simulink model "sfWindTurbine"  (R2025b)
settings: Solver=ode23t  StartTime=0.0  StopTime=simT  RelTol=1e-3  AbsTol=1e-3
PreLoadFcn:
  | load sfWindTurbineParameters.mat
values from neighbouring files (symbols this model uses):
  actuatorRampRate = 20    [sfWindTurbineParameters.mat]
  airDensity = 1.15    [sfWindTurbineParameters.mat]
  carrierShaftInertia = 10    [sfWindTurbineParameters.mat]
  controllerTimeConstant = 2    [sfWindTurbineParameters.mat]
  cp = [1e-05 1e-05 1e-05 1e-05 1e-05 1e-05 1e-05 1e-05 1e-05 1e-05 1e-05 1e-05 ... (3015 elements, 15x201)]    [sfWindTurbineParameters.mat]
  Derating = [12 13 14 15 16 17 18 19 20 1 4 7 ... (18 elements, 9x2)]    [sfWindTurbineParameters.mat]
  firstStepTeethRatio = 3.05    [sfWindTurbineParameters.mat]
  generatorEfficiency = 100    [sfWindTurbineParameters.mat]
  generatorInertia = 200    [sfWindTurbineParameters.mat]
  generatorLumpedInductance = 0.0001916    [sfWindTurbineParameters.mat]
  generatorLumpedResistance = 0.0027    [sfWindTurbineParameters.mat]
  gridFrequency = 60    [sfWindTurbineParameters.mat]
  iGenerationGain = 1    [sfWindTurbineParameters.mat]
  maxPitchAngle = 25    [sfWindTurbineParameters.mat]
  minPitchAngle = 1    [sfWindTurbineParameters.mat]
  mpptOmega = [502.335 613.965 753.5025 865.1325 1004.67 1116.3 1200.0225 1200.0225 1200.0225]    [sfWindTurbineParameters.mat]
  mpptPower = [0.0596400180021 0.116487570967 0.201285060757 0.319665137738 0.477120144017 0.679427108153 0.931130687114 1.22525336077 1.55330342875]    [sfWindTurbineParameters.mat]
  mpptWindSpeed = [4 5 6 7 8 9 10 11 12]    [sfWindTurbineParameters.mat]
  pGenerationGain = 100    [sfWindTurbineParameters.mat]
  pGeneratorBrakeLimit = 0.5    [sfWindTurbineParameters.mat]
  pitch = [1 3 5 7 9 11 13 15 17 19 21 23 ... (15 elements, 1x15)]    [sfWindTurbineParameters.mat]
  pitchBrakeAngle = 95    [sfWindTurbineParameters.mat]
  ringSunTeethRatio = 6    [sfWindTurbineParameters.mat]
  rotorBladeInertia = 3963845    [sfWindTurbineParameters.mat]
  secondStepTeethRatio = 3.05    [sfWindTurbineParameters.mat]
  simT = 800    [sfWindTurbineParameters.mat]
  stepShaftInertia = 10    [sfWindTurbineParameters.mat]
  TSR = [0 0.1 0.2 0.3 0.4 0.5 0.6 0.7 0.8 0.9 1 1.1 ... (201 elements, 1x201)]    [sfWindTurbineParameters.mat]
  turbineRadius = 35.25    [sfWindTurbineParameters.mat]
  turbineRatedPower = 1.5    [sfWindTurbineParameters.mat]
  vWindCutOut = 20    [sfWindTurbineParameters.mat]
  wAtGeneratorRatedPower = 1227.93    [sfWindTurbineParameters.mat]
  wGeneratorBrakeLimit = 0.5    [sfWindTurbineParameters.mat]
libraries: simulink x6, slpidlib x1, SignalEditorBlockLib x1
Description:
  | Wind Turbine
settings Model: PauseTimes=599  Creator=The MathWorks, Inc.  LastModifiedBy=The MathWorks, Inc.
settings SolverCC: AutoScaleAbsTol=off  MaxConsecutiveMinStep=5  AlgebraicLoopSolver=TrustRegion  MaxZcPerStep=1.0
settings DataIOCC: SaveOutput=off  DSMLogging=off  SaveTime=off  ReturnWorkspaceOutputs=off  SignalLoggingName=logsout_sscv_wind_turbine
settings OptimizationCC: ReuseModelBlockBuffer=off
settings DebuggingCC: UnconnectedInputMsg=warning  UnconnectedOutputMsg=warning  UnconnectedLineMsg=warning
settings ModelReferenceCC: EnableRefExpFcnMdlSchedulingChecks=on
settings RTWCC: GPUComputeCapability=3.5  DLArmComputeVersion=19.05
settings SimscapeCC: SimscapeLogType=all  SimscapeLogSimulationStatistics=on  SimscapeLogName=simlog_sscv_wind_turbine  SimscapeLogDataHistory=10000000.0
settings ConfigComp: PLC_FoldFBCallOutputVar=off  PLC_RemoveUnusedSSMethodCallArguments=off  PLC_ActiveTab=0.0  PLC_UseCallOutputArgSyntax=off  PLC_TargetIDE=codesys35  PLC_EnableUnsignedAndDoubleTypes=off  PLC_RollThreshold=5.0  PLC_EnableUDTSplitting=off  PLC_MultiTBSigbuilderTimeRange=off  PLC_MaxFieldsInUDT=500.0  PLC_EnableStringLiteralTB=on  PLC_InlineEnumCastFunction=off  PLC_Enable64bitIntSupport=off  PLC_RTWMaxIdLength=31.0

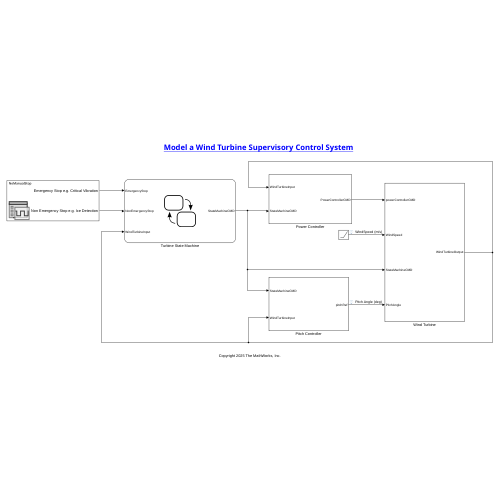
[thumbnail: Simulink's stored preview of the top-level diagram]
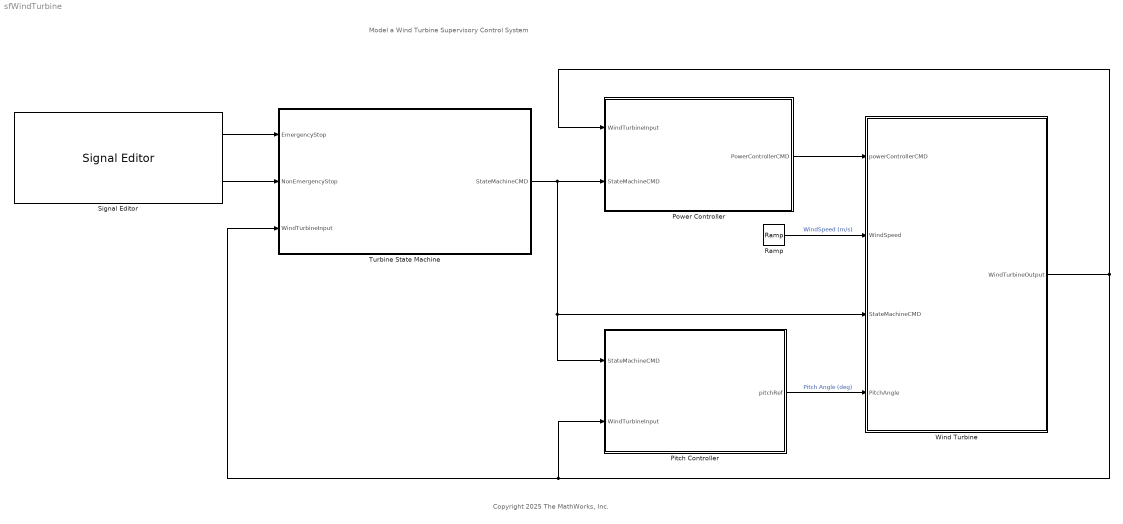
== system sfWindTurbine ==
  note: Model a Wind Turbine Supervisory Control System
  note: Copyright 2025 The MathWorks, Inc.
  Pitch Controller : Subsystem
  Power Controller : Subsystem
  Ramp : simulink/Sources/Ramp  slope=(vWindCutOut+2)/simT  start=0  InitialOutput=0
  Signal Editor : SignalEditorBlockLib/Signal Editor  FileName=ManualStopSignal.mat  ActiveScenario=NoManualStop  ActiveSignal=Emergency Stop e.g. Critical Vibration  IsBus=off  OutputBusObjectStr=Bus: BusObject  SampleTime=0  Interpolate=off  ZeroCross=off  OutputAfterFinalValue=Setting to zero  Unit=inherit  PreserveSignalName=on  ApplySigPropsToAllScenarios=on  ApplySigPropsToAllSignals=off  SignalPropertySource=Dialog parameters
  Turbine State Machine : Stateflow chart  TreatAsAtomicUnit=on
  Wind Turbine : Subsystem
  wires:
  Turbine State Machine/1(StateMachineCMD) -> Pitch Controller/1(StateMachineCMD), Wind Turbine/3(StateMachineCMD), Power Controller/2(StateMachineCMD)
  Pitch Controller/1(pitchRef) -> Wind Turbine/4(PitchAngle)  "Pitch Angle (deg)"
  Ramp/1 -> Wind Turbine/2(WindSpeed)  "WindSpeed (m/s)"
  Power Controller/1(PowerControllerCMD) -> Wind Turbine/1(powerControllerCMD)
  Wind Turbine/1(WindTurbineOutput) -> Power Controller/1(WindTurbineInput), Pitch Controller/2(WindTurbineInput), Turbine State Machine/3(WindTurbineInput)
  Signal Editor/1 -> Turbine State Machine/1(EmergencyStop)
  Signal Editor/2 -> Turbine State Machine/2(NonEmergencyStop)

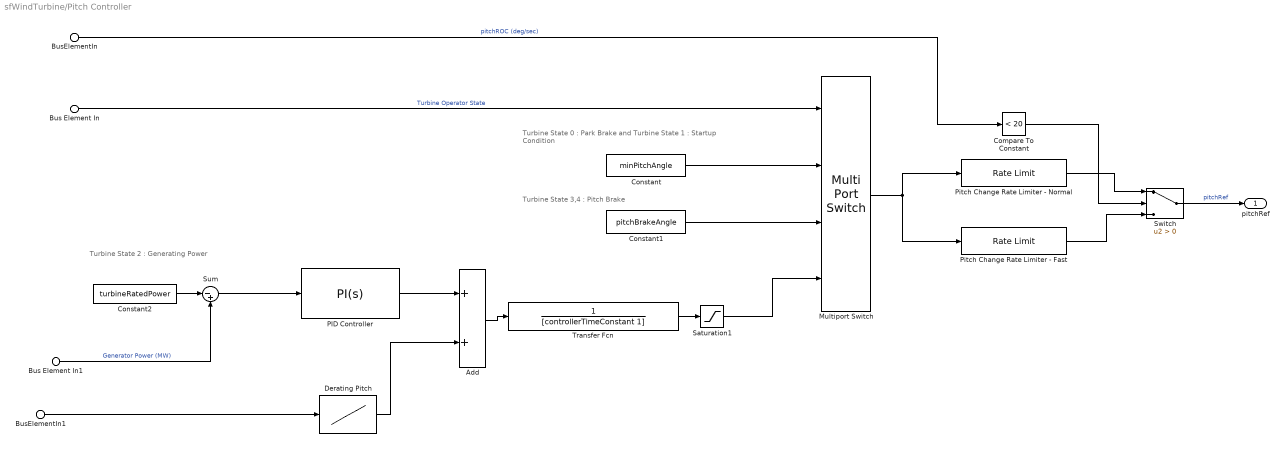
== system sfWindTurbine/Pitch Controller ==
  note: Turbine State 2 : Generating Power
  note: Turbine State 0 : Park Brake and
      | Turbine State 1 : Startup Condition
  note: Turbine State 3,4 : Pitch Brake
  Bus Element In : Inport  PortName=StateMachineCMD  Element=turbineState
  BusElementIn : Inport  PortName=StateMachineCMD  Element=pitchROC
  Bus Element In1 : Inport  Port=2  PortName=WindTurbineInput  Element=GeneratorPower
  BusElementIn1 : Inport  Port=2  PortName=WindTurbineInput  Element=WindSpeed
  Add : Sum  Inputs=2
  Compare To Constant : simulink/Logic and Bit Operations/Compare To Constant  relop=<  const=20  OutDataTypeStr=boolean
  Constant : Constant  Value=minPitchAngle
  Constant1 : Constant  Value=pitchBrakeAngle
  Constant2 : Constant  Value=turbineRatedPower
  Derating Pitch : Lookup_n-D  NumberOfTableDimensions=1  BreakpointsForDimension1=Derating(:,1)  Table=Derating(:,2)-minPitchAngle  InternalRulePriority=Speed  RndMeth=Simplest
  Multiport Switch : MultiPortSwitch  DataPortOrder=Specify indices  DataPortIndices={[0,1],[3,4],2}  SaturateOnIntegerOverflow=off  InputSameDT=off
  PID Controller : slpidlib/PID Controller  Controller=PI  Form=Parallel  TimeDomain=Continuous-time  UseExternalTs=off  SampleTime=-1  IntegratorMethod=Forward Euler  FilterMethod=Forward Euler  ControllerParametersSource=internal  P=pGenerationGain  I=iGenerationGain  UseKiTs=off  D=0  UseExternalDerivativeSource=off  N=100  UseFilter=on  TunerSelectOption=Transfer Function Based (PID Tuner App)  InitialConditionSource=internal  InitialConditionForIntegrator=1  InitialConditionForFilter=0  DifferentiatorICPrevScaledInput=0  ExternalReset=none  TrackingMode=off  Kt=1  LimitOutput=on  SatLimitsSource=internal  UpperSaturationLimit=maxPitchAngle  LowerSaturationLimit=minPitchAngle  LinearizeAsGain=on  AntiWindupMode=clamping  Kb=1  LimitIntegrator=off  UpperIntegratorSaturationLimit=inf  LowerIntegratorSaturationLimit=-inf  POutMin=[]  POutMax=[]  IOutMin=[]  IOutMax=[]  DOutMin=[]  DOutMax=[]  NOutMin=[]  NOutMax=[]  SumOutMin=[]  SumOutMax=[]  SaturationOutMin=[]  SaturationOutMax=[]  PParamMin=[]  PParamMax=[]  IParamMin=[]  IParamMax=[]  DParamMin=[]  DParamMax=[]  NParamMin=[]  NParamMax=[]  KbParamMin=[]  KbParamMax=[]  KtParamMin=[]  KtParamMax=[]  KbOutMin=[]  KbOutMax=[]  KtOutMin=[]  KtOutMax=[]  IntegratorOutMin=[]  IntegratorOutMax=[]  FilterOutMin=[]  FilterOutMax=[]  SumI1OutMin=[]  SumI1OutMax=[]  SumI2OutMin=[]  SumI2OutMax=[]  SumI3OutMin=[]  SumI3OutMax=[]  SumI4OutMin=[]  SumI4OutMax=[]  SumDOutMin=[]  SumDOutMax=[]  DifferentiatorOutMin=[]  DifferentiatorOutMax=[]  FilterDiffOutCoefMin=[]  FilterDiffOutCoefMax=[]  ReciprocalOutMin=[]  ReciprocalOutMax=[]  SumDenOutMin=[]  SumDenOutMax=[]  SumNumOutMin=[]  SumNumOutMax=[]  DivideOutMin=[]  DivideOutMax=[]  UdiffTsProdOutMin=[]  UdiffTsProdOutMax=[]  NTsProdOutMin=[]  NTsProdOutMax=[]  UintegralTsProdOutMin=[]  UintegralTsProdOutMax=[]  UngainTsProdOutMin=[]  UngainTsProdOutMax=[]  ClampingZeroOutDataTypeStr=Inherit: Inherit via back propagation  ClampingZeroOutMin=[]  ClampingZeroOutMax=[]  FilterDenConstantOutDataTypeStr=Inherit: Inherit via back propagation  FilterDenConstantOutMin=[]  FilterDenConstantOutMax=[]  PCopyOutDataTypeStr=Inherit: Inherit via back propagation  PCopyOutMin=[]  PCopyOutMax=[]  NCopyOutDataTypeStr=Inherit: Inherit via back propagation  NCopyOutMin=[]  NCopyOutMax=[]  IntegratorContinuousStateAttributes=''  IntegratorStateMustResolveToSignalObject=off  IntegratorRTWStateStorageClass=Auto  FilterContinuousStateAttributes=''  FilterStateMustResolveToSignalObject=off  FilterRTWStateStorageClass=Auto  ParallelPVariant=InternalParameters  IdealPVariant=Disabled  IVariant=InternalParameters  DVariant=Disabled  IntegratorVariant=Continuous  SatVariant=Enabled  AWVariant=ContClampingParallel  PCopyVariant=Disabled  TRVariant=Disabled  FdbkBlocksVariant=Forward  IdealPFdbkVariant=Disabled  SatFdbkVariant=Disabled  DerivativeFilterVariant=Disabled  NVariant=Disabled  NCopyVariant=Disabled_SignalSpec  FilterICVariant=Disabled  IntegratorICVariant=InternalICs  ExternalResetVariant=Disabled  TRSumVariant=Passthrough  SumFdbkVariant=Disabled  SumVariant=Sum_PI  TsampFilterVariant=InternalTs  TsampNgainVariant=Passthrough  TsampIntegralVariant=Disabled_SignalSpec  ExternalSaturationOutDataTypeStr=Inherit: Same as second input  DerivativeSourceVariant=Disabled  PreIntVariant=InternalPreInt
      settings: AttributesFormatString=|
      | %<AntiWindupMode>
      | %<I>
      | %<P>
      | %<UpperSaturationLimit>
      | %<LowerSaturationLimit>
  Pitch Change Rate Limiter - Fast : RateLimiter  RisingSlewLimit=actuatorRampRate  FallingSlewLimit=-actuatorRampRate  SampleTimeMode=inherited
  Pitch Change Rate Limiter - Normal : RateLimiter  RisingSlewLimit=actuatorRampRate/4  FallingSlewLimit=-actuatorRampRate/4  SampleTimeMode=inherited
  Saturation1 : Saturate  UpperLimit=maxPitchAngle  LowerLimit=minPitchAngle
  Sum : Sum  Inputs=|-+
  Switch : Switch  Criteria=u2 > Threshold  SaturateOnIntegerOverflow=off  InputSameDT=off
  Transfer Fcn : TransferFcn  Denominator=[controllerTimeConstant 1]
  pitchRef : Outport
  wires:
  Pitch Change Rate Limiter - Normal/1 -> Switch/1
  Derating Pitch/1 -> Add/2
  Compare To Constant/1 -> Switch/2
  Pitch Change Rate Limiter - Fast/1 -> Switch/3
  Multiport Switch/1 -> Pitch Change Rate Limiter - Fast/1, Pitch Change Rate Limiter - Normal/1
  Constant/1 -> Multiport Switch/2
  Saturation1/1 -> Multiport Switch/4
  PID Controller/1 -> Add/1
  Constant1/1 -> Multiport Switch/3
  Transfer Fcn/1 -> Saturation1/1
  Add/1 -> Transfer Fcn/1
  Constant2/1 -> Sum/1
  Sum/1 -> PID Controller/1
  Switch/1 -> pitchRef/1  "pitchRef"
  BusElementIn/1 -> Compare To Constant/1  "pitchROC (deg/sec)"
  Bus Element In1/1 -> Sum/2  "Generator Power (MW)"
  Bus Element In/1 -> Multiport Switch/1  "Turbine Operator State"
  BusElementIn1/1 -> Derating Pitch/1

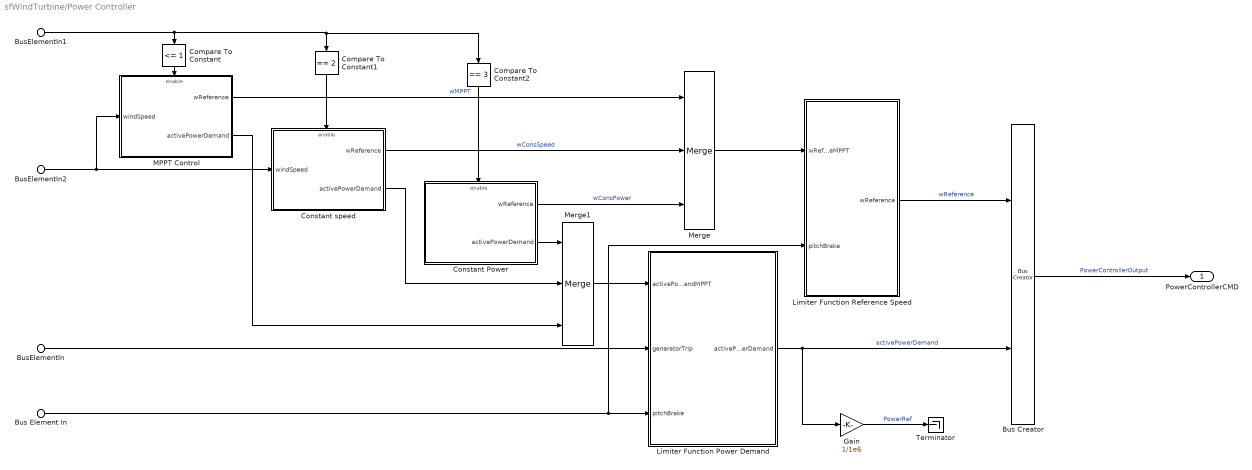
== system sfWindTurbine/Power Controller ==
  BusElementIn2 : Inport  PortName=WindTurbineInput  Element=WindSpeed
  Bus Element In : Inport  Port=2  PortName=StateMachineCMD  Element=pitchBrake
  BusElementIn : Inport  Port=2  PortName=StateMachineCMD  Element=generatorTrip
  BusElementIn1 : Inport  Port=2  PortName=StateMachineCMD  Element=powerGenState
  Bus Creator : BusCreator  Inputs=2
  Compare To Constant : simulink/Logic and Bit Operations/Compare To Constant  relop=<=  const=1  OutDataTypeStr=boolean
  Compare To Constant1 : simulink/Logic and Bit Operations/Compare To Constant  relop===  const=2  OutDataTypeStr=boolean
  Compare To Constant2 : simulink/Logic and Bit Operations/Compare To Constant  relop===  const=3  OutDataTypeStr=boolean
  Constant Power : Subsystem
  Constant speed : Subsystem
  Gain : Gain  Gain=1/1e6
  Limiter Function Power Demand : Subsystem
  Limiter Function Reference Speed : Subsystem
  MPPT Control : Subsystem
  Merge : Merge  Inputs=3
  Merge1 : Merge  Inputs=3
  Terminator : Terminator
  PowerControllerCMD : Outport
  wires:
  Bus Creator/1 -> PowerControllerCMD/1  "PowerControllerOutput"
  Limiter Function Power Demand/1(activePowerDemand) -> Gain/1, Bus Creator/2  "activePowerDemand"
  Merge/1 -> Limiter Function Reference Speed/1(wReferenceMPPT)
  Compare To Constant/1 -> MPPT Control/Enable
  Compare To Constant2/1 -> Constant Power/Enable
  Bus Element In/1 -> Limiter Function Reference Speed/2(pitchBrake), Limiter Function Power Demand/3(pitchBrake)
  BusElementIn/1 -> Limiter Function Power Demand/2(generatorTrip)
  Constant speed/1(wReference) -> Merge/2  "wConsSpeed"
  Merge1/1 -> Limiter Function Power Demand/1(activePowerDemandMPPT)
  Constant speed/2(activePowerDemand) -> Merge1/2
  Constant Power/2(activePowerDemand) -> Merge1/1
  BusElementIn1/1 -> Compare To Constant2/1, Compare To Constant1/1, Compare To Constant/1
  Constant Power/1(wReference) -> Merge/3  "wConsPower"
  Limiter Function Reference Speed/1(wReference) -> Bus Creator/1  "wReference"
  Gain/1 -> Terminator/1  "PowerRef"
  Compare To Constant1/1 -> Constant speed/Enable
  MPPT Control/1(wReference) -> Merge/1  "wMPPT"
  MPPT Control/2(activePowerDemand) -> Merge1/3
  BusElementIn2/1 -> MPPT Control/1(windSpeed), Constant speed/1(windSpeed)

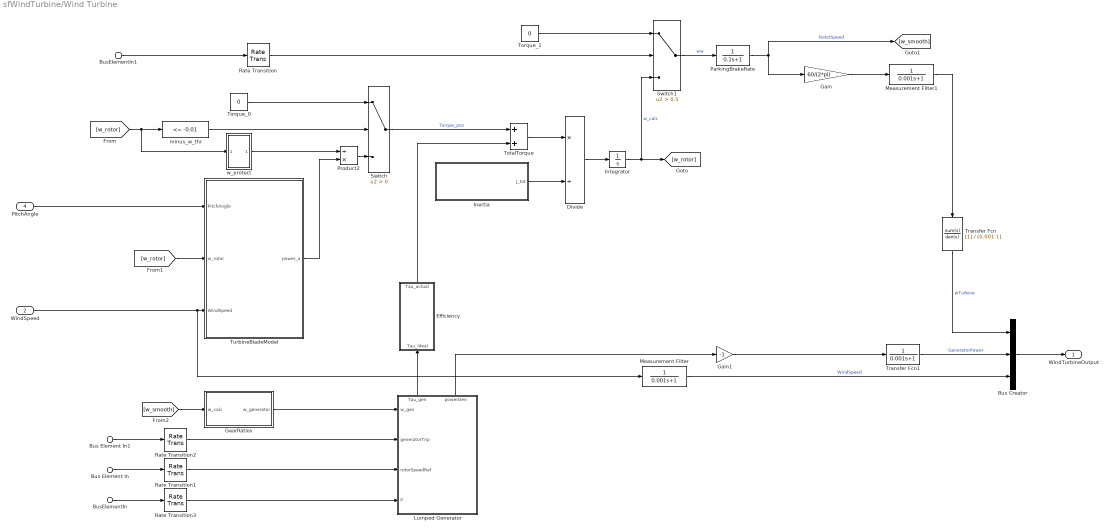
== system sfWindTurbine/Wind Turbine ==
  Bus Element In : Inport  PortName=powerControllerCMD  Element=wReference
  BusElementIn : Inport  PortName=powerControllerCMD  Element=activePowerDemand
  WindSpeed : Inport  Port=2
  Bus Element In1 : Inport  Port=3  PortName=StateMachineCMD  Element=generatorTrip
  BusElementIn1 : Inport  Port=3  PortName=StateMachineCMD  Element=parkingBrake
  PitchAngle : Inport  Port=4
  Bus Creator : BusCreator  Inputs=3
  Divide : Product  Inputs=*/
  Efficiency : Subsystem
  Gain : Gain  Gain=60/(2*pi)
  Gain1 : Gain  Gain=-1
  GearRatios : Subsystem
  Inertia : Subsystem
  Integrator : Integrator  InitialCondition=0.01
  Lumped Generator : Subsystem  mask{ratedPower=turbineRatedPower, gridFreq=gridFrequency, genResistor=generatorLumpedResistance, genInductance=generatorLumpedInductance, genEfficiency=generatorEfficiency, ratedSpeed=wAtGeneratorRatedPower}
      mask prompts: ratedPower "Rated power (MW)"; gridFreq "Grid frequency (Hz)"; genResistor "Electrical generator lumped resistance (Ohm)"; genInductance "Electrical generator lumped leakage inductance (H)"; genEfficiency "Electrical generator effficiency"; ratedSpeed "Wind turbine speed at rated wind speed (rpm)"
      settings: PortSchema="{\"entries\":[{\"content\":{\"sides\":[{\"content\":{},\"type\":\"ConnectorPlacement.EquallySpacedRectSide\",\"uuid\":\"600b86f2-4f8f-493b-ad26-1faa8bb85470\"},{\"content\":{\"connectorIds\":[\"Out1\",\"Out2\"],\"side\":\"RIGHT\"},\"type\":\"ConnectorPlacement.EquallySpacedRectSide\",\"uuid\":\"9e1649b7-9973-42e8-ab8f-93eff55c3d74\"},{\"content\":{\"connectorIds\":[\"In1\",\"In2\",\"In3\",\"In4\"],\"side\":\"TOP\"},\"type\":\"ConnectorPlacement.EquallySpacedRectSide\",\"uuid\":\"66dc1112-3744-4fa2-a344-a6dc92e314fc\"},{\"content\":{\"side\":\"BOTTOM\"},\"type\":\"ConnectorPlacement.EquallySpacedRectSide\",\"uuid\":\"0ba4da35-be81-423d-9ede-c806323f0c4b\"}]},\"type\":\"ConnectorPlacement.EquallySpacedConnector\",\"uuid\":\"3b2d2e6e-f4ee-4b4b-84c0-3ef19b29de27\"}],\"packageUris\":[\"http://schema.mathworks.com/mf0/Connector/R2020b\"],\"version\":\"1.0\"}"
      mask Display: disp('Lumped Generator');
  Measurement Filter : TransferFcn  Denominator=[0.001 1]
  Measurement Filter1 : TransferFcn  Denominator=[0.001 1]
  ParkingBrakeRate : TransferFcn  Denominator=[0.1 1]
  Product2 : Product  Inputs=/*
  Rate Transition{,1..3} (4 alike) : RateTransition
  Switch : Switch  Criteria=u2 > Threshold  SaturateOnIntegerOverflow=off  InputSameDT=off
  Switch1 : Switch  Criteria=u2 > Threshold  Threshold=0.5  SaturateOnIntegerOverflow=off  InputSameDT=off
  Torque_0 : Constant  Value=0
  Torque_1 : Constant  Value=0
  TotalTorque : Sum
  Transfer Fcn : TransferFcn  Denominator=[0.001 1]
  Transfer Fcn1 : TransferFcn  Denominator=[0.001 1]
  TurbineBladeModel : Subsystem
  minus_w_thr : simulink/Logic and Bit Operations/Compare To Constant  relop=<=  const=-0.01  OutDataTypeStr=boolean
  w_protect : Subsystem
  WindTurbineOutput : Outport
  wires:
  WindSpeed/1 -> Measurement Filter/1, TurbineBladeModel/3(WindSpeed)
  minus_w_thr/1 -> Switch/2
  Switch1/1 -> ParkingBrakeRate/1  "ww"
  Lumped Generator/2(powerGen) -> Gain1/1
  [w_rotor] -> w_protect/1(In1), minus_w_thr/1
  ParkingBrakeRate/1 -> Gain/1, [w_smooth]  "RototSpeed"
  Torque_1/1 -> Switch1/1
  Torque_0/1 -> Switch/1
  Efficiency/1(Tau_actual) -> TotalTorque/2
  [w_rotor] -> TurbineBladeModel/2(w_rotor)
  w_protect/1(Out1) -> Product2/1
  PitchAngle/1 -> TurbineBladeModel/1(PitchAngle)
  [w_smooth] -> GearRatios/1(w_calc)
  Divide/1 -> Integrator/1
  Lumped Generator/1(Tau_gen) -> Efficiency/1(Tau_Ideal)
  GearRatios/1(w_generator) -> Lumped Generator/4(w_gen)
  Inertia/1(J_tot) -> Divide/2
  Switch/1 -> TotalTorque/1  "Torque_pos"
  Integrator/1 -> Switch1/3, [w_rotor]  "w_calc"
  Product2/1 -> Switch/3
  TurbineBladeModel/1(power_a) -> Product2/2
  TotalTorque/1 -> Divide/1
  Measurement Filter/1 -> Bus Creator/3  "WindSpeed"
  Bus Creator/1 -> WindTurbineOutput/1
  Rate Transition/1 -> Switch1/2
  Rate Transition1/1 -> Lumped Generator/2(rotorSpeedRef)
  Rate Transition2/1 -> Lumped Generator/3(generatorTrip)
  Rate Transition3/1 -> Lumped Generator/1(P)
  Gain/1 -> Measurement Filter1/1
  Measurement Filter1/1 -> Transfer Fcn/1
  Gain1/1 -> Transfer Fcn1/1
  Transfer Fcn1/1 -> Bus Creator/2  "GeneratorPower"
  Transfer Fcn/1 -> Bus Creator/1  "wTurbine"
  BusElementIn1/1 -> Rate Transition/1
  BusElementIn/1 -> Rate Transition3/1
  Bus Element In/1 -> Rate Transition1/1
  Bus Element In1/1 -> Rate Transition2/1

== system sfWindTurbine/Power Controller/Constant Power ==
  Enable : EnablePort  StatesWhenEnabling=reset
  Constant : Constant  Value=max(mpptOmega)
  Constant1 : Constant  Value=turbineRatedPower
  MW to W : Gain  Gain=1e6
  wReference : Outport
  activePowerDemand : Outport  Port=2
  wires:
  Constant/1 -> wReference/1
  MW to W/1 -> activePowerDemand/1
  Constant1/1 -> MW to W/1

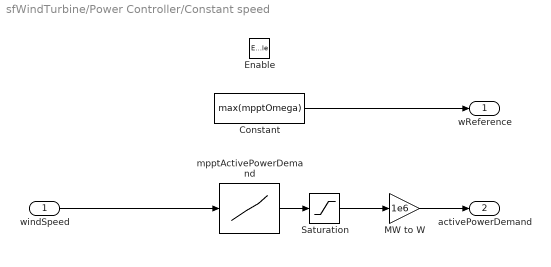
== system sfWindTurbine/Power Controller/Constant speed ==
  windSpeed : Inport
  Enable : EnablePort  StatesWhenEnabling=reset
  Constant : Constant  Value=max(mpptOmega)
  MW to W : Gain  Gain=1e6
  Saturation : Saturate  UpperLimit=turbineRatedPower  LowerLimit=0
  mpptActivePowerDemand : Lookup_n-D  NumberOfTableDimensions=1  BreakpointsForDimension1=mpptWindSpeed  Table=mpptPower  ExtrapMethod=Clip  InternalRulePriority=Speed  RndMeth=Simplest
  wReference : Outport
  activePowerDemand : Outport  Port=2
  wires:
  mpptActivePowerDemand/1 -> Saturation/1
  windSpeed/1 -> mpptActivePowerDemand/1
  Constant/1 -> wReference/1
  MW to W/1 -> activePowerDemand/1
  Saturation/1 -> MW to W/1

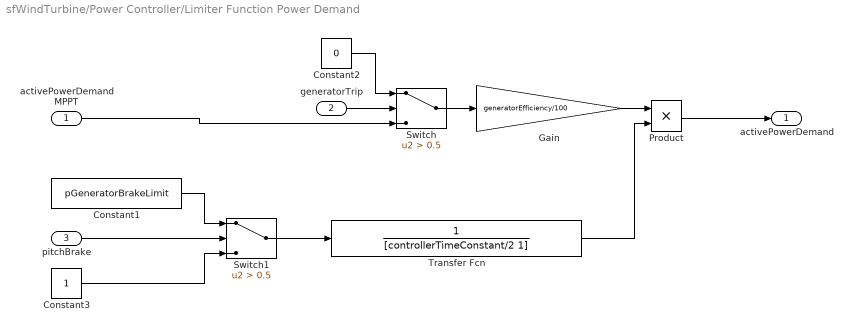
== system sfWindTurbine/Power Controller/Limiter Function Power Demand ==
  activePowerDemandMPPT : Inport
  generatorTrip : Inport  Port=2
  pitchBrake : Inport  Port=3
  Constant1 : Constant  Value=pGeneratorBrakeLimit
  Constant2 : Constant  Value=0
  Constant3 : Constant
  Gain : Gain  Gain=generatorEfficiency/100
  Product : Product
  Switch : Switch  Criteria=u2 > Threshold  Threshold=0.5  SaturateOnIntegerOverflow=off  InputSameDT=off
  Switch1 : Switch  Criteria=u2 > Threshold  Threshold=0.5  SaturateOnIntegerOverflow=off  InputSameDT=off
  Transfer Fcn : TransferFcn  Denominator=[controllerTimeConstant/2 1]
  activePowerDemand : Outport
  wires:
  generatorTrip/1 -> Switch/2
  Switch/1 -> Gain/1
  Constant2/1 -> Switch/1
  activePowerDemandMPPT/1 -> Switch/3
  pitchBrake/1 -> Switch1/2
  Constant3/1 -> Switch1/3
  Constant1/1 -> Switch1/1
  Gain/1 -> Product/1
  Switch1/1 -> Transfer Fcn/1
  Product/1 -> activePowerDemand/1
  Transfer Fcn/1 -> Product/2

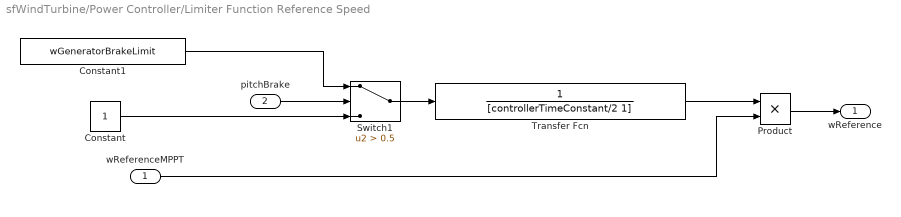
== system sfWindTurbine/Power Controller/Limiter Function Reference Speed ==
  wReferenceMPPT : Inport
  pitchBrake : Inport  Port=2
  Constant : Constant
  Constant1 : Constant  Value=wGeneratorBrakeLimit
  Product : Product
  Switch1 : Switch  Criteria=u2 > Threshold  Threshold=0.5  SaturateOnIntegerOverflow=off  InputSameDT=off
  Transfer Fcn : TransferFcn  Denominator=[controllerTimeConstant/2 1]
  wReference : Outport
  wires:
  pitchBrake/1 -> Switch1/2
  Constant1/1 -> Switch1/1
  wReferenceMPPT/1 -> Product/2
  Constant/1 -> Switch1/3
  Product/1 -> wReference/1
  Transfer Fcn/1 -> Product/1
  Switch1/1 -> Transfer Fcn/1

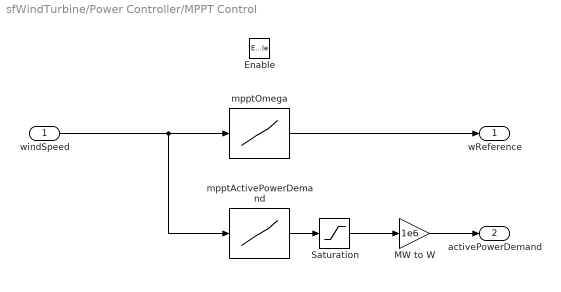
== system sfWindTurbine/Power Controller/MPPT Control ==
  windSpeed : Inport
  Enable : EnablePort  StatesWhenEnabling=reset
  MW to W : Gain  Gain=1e6
  Saturation : Saturate  UpperLimit=turbineRatedPower  LowerLimit=0
  mpptActivePowerDemand : Lookup_n-D  NumberOfTableDimensions=1  BreakpointsForDimension1=mpptWindSpeed  Table=mpptPower  ExtrapMethod=Clip  InternalRulePriority=Speed  RndMeth=Simplest
  mpptOmega : Lookup_n-D  NumberOfTableDimensions=1  BreakpointsForDimension1=mpptWindSpeed  Table=mpptOmega  ExtrapMethod=Clip  InternalRulePriority=Speed  RndMeth=Simplest
  wReference : Outport
  activePowerDemand : Outport  Port=2
  wires:
  mpptActivePowerDemand/1 -> Saturation/1
  windSpeed/1 -> mpptActivePowerDemand/1, mpptOmega/1
  mpptOmega/1 -> wReference/1
  MW to W/1 -> activePowerDemand/1
  Saturation/1 -> MW to W/1

== system sfWindTurbine/Wind Turbine/Efficiency ==
  Tau_Ideal : Inport
  Efficiency : Gain  Gain=1/0.83
  ratio1 : Gain  Gain=ringSunTeethRatio
  ratio2 : Gain  Gain=firstStepTeethRatio
  ratio3 : Gain  Gain=secondStepTeethRatio
  Tau_actual : Outport
  wires:
  ratio1/1 -> ratio2/1
  ratio3/1 -> Efficiency/1
  ratio2/1 -> ratio3/1
  Tau_Ideal/1 -> ratio1/1
  Efficiency/1 -> Tau_actual/1

== system sfWindTurbine/Wind Turbine/GearRatios ==
  w_calc : Inport
  ratio1 : Gain  Gain=ringSunTeethRatio
  ratio2 : Gain  Gain=-firstStepTeethRatio
  ratio3 : Gain  Gain=secondStepTeethRatio
  w_generator : Outport
  wires:
  ratio1/1 -> ratio2/1
  ratio3/1 -> w_generator/1  "w_generator"
  ratio2/1 -> ratio3/1
  w_calc/1 -> ratio1/1

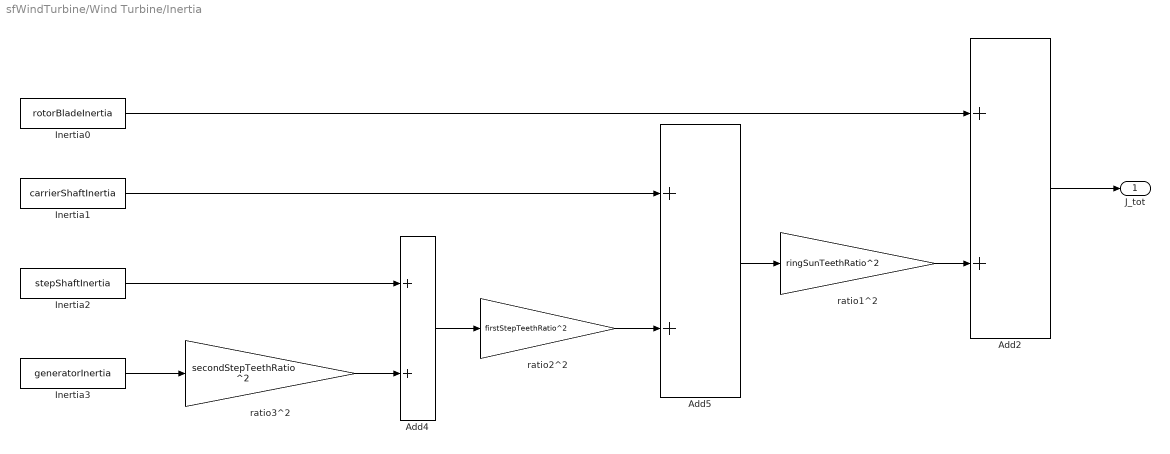
== system sfWindTurbine/Wind Turbine/Inertia ==
  Add2 : Sum
  Add4 : Sum
  Add5 : Sum
  Inertia0 : Constant  Value=rotorBladeInertia
  Inertia1 : Constant  Value=carrierShaftInertia
  Inertia2 : Constant  Value=stepShaftInertia
  Inertia3 : Constant  Value=generatorInertia
  ratio1^2 : Gain  Gain=ringSunTeethRatio^2
  ratio2^2 : Gain  Gain=firstStepTeethRatio^2
  ratio3^2 : Gain  Gain=secondStepTeethRatio ^2
  J_tot : Outport
  wires:
  ratio1^2/1 -> Add2/2
  Inertia2/1 -> Add4/1
  Inertia0/1 -> Add2/1
  Inertia3/1 -> ratio3^2/1
  Inertia1/1 -> Add5/1
  ratio2^2/1 -> Add5/2
  ratio3^2/1 -> Add4/2
  Add2/1 -> J_tot/1
  Add4/1 -> ratio2^2/1
  Add5/1 -> ratio1^2/1

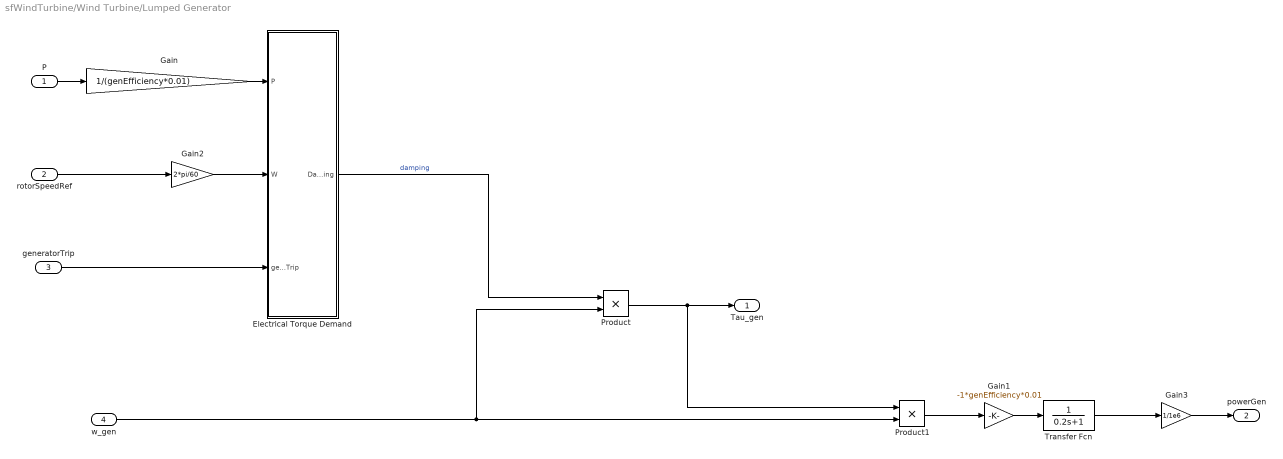
== system sfWindTurbine/Wind Turbine/Lumped Generator ==
  P : Inport
  rotorSpeedRef : Inport  Port=2
  generatorTrip : Inport  Port=3
  w_gen : Inport  Port=4
  Electrical Torque Demand : Subsystem
  Gain : Gain  Gain=1/(genEfficiency*0.01)
  Gain1 : Gain  Gain=-1*genEfficiency*0.01
  Gain2 : Gain  Gain=2*pi/60
  Gain3 : Gain  Gain=1/1e6
  Product : Product
  Product1 : Product
  Transfer Fcn : TransferFcn  Denominator=[0.2 1]
  Tau_gen : Outport
  powerGen : Outport  Port=2
  wires:
  P/1 -> Gain/1
  rotorSpeedRef/1 -> Gain2/1
  Electrical Torque Demand/1(Damping) -> Product/1  "damping"
  Gain2/1 -> Electrical Torque Demand/2(W)
  Gain/1 -> Electrical Torque Demand/1(P)
  Gain1/1 -> Transfer Fcn/1
  generatorTrip/1 -> Electrical Torque Demand/3(generatorTrip)
  Transfer Fcn/1 -> Gain3/1
  Gain3/1 -> powerGen/1
  w_gen/1 -> Product/2, Product1/2
  Product/1 -> Product1/1, Tau_gen/1
  Product1/1 -> Gain1/1

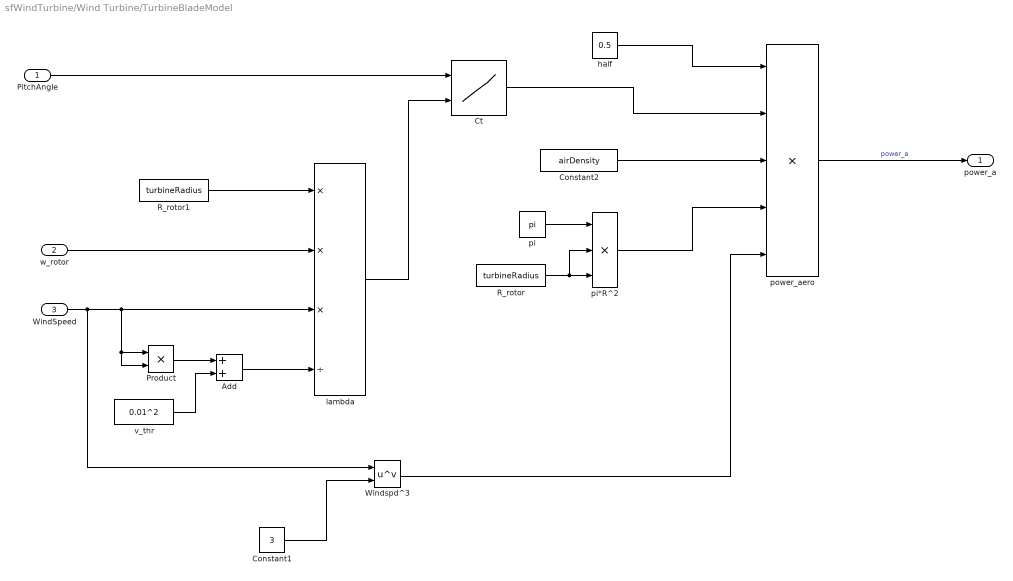
== system sfWindTurbine/Wind Turbine/TurbineBladeModel ==
  PitchAngle : Inport
  w_rotor : Inport  Port=2
  WindSpeed : Inport  Port=3
  Add : Sum
  Constant1 : Constant  Value=3
  Constant2 : Constant  Value=airDensity
  Ct : Lookup_n-D  BreakpointsForDimension1=pitch  BreakpointsForDimension2=TSR  Table=cp  ExtrapMethod=Clip  UseLastTableValue=on  InternalRulePriority=Speed  RndMeth=Simplest
      settings: InputPortMap=u0,u1
  Product : Product
  R_rotor : Constant  Value=turbineRadius
  R_rotor1 : Constant  Value=turbineRadius
  Windspd^3 : Math  Operator=pow
  half : Constant  Value=0.5
  lambda : Product  Inputs=***/
  pi : Constant  Value=pi
  pi*R^2 : Product  Inputs=3
  power_aero : Product  Inputs=5
  v_thr : Constant  Value=0.01^2
  power_a : Outport
  wires:
  pi*R^2/1 -> power_aero/4
  WindSpeed/1 -> Windspd^3/1, Product/2, Product/1, lambda/3
  Windspd^3/1 -> power_aero/5
  Constant1/1 -> Windspd^3/2
  lambda/1 -> Ct/2
  R_rotor1/1 -> lambda/1
  R_rotor/1 -> pi*R^2/3, pi*R^2/2
  half/1 -> power_aero/1
  v_thr/1 -> Add/2
  Add/1 -> lambda/4
  Product/1 -> Add/1
  Constant2/1 -> power_aero/3
  Ct/1 -> power_aero/2
  pi/1 -> pi*R^2/1
  w_rotor/1 -> lambda/2
  PitchAngle/1 -> Ct/1
  power_aero/1 -> power_a/1  "power_a"

== system sfWindTurbine/Wind Turbine/w_protect ==
  In1 : Inport
  Add1 : Sum
  Product1 : Product
  Saturation : Saturate  UpperLimit=inf  LowerLimit=-0.01
  Sqrt : Sqrt
  w_thr : Constant  Value=0.01^2
  Out1 : Outport
  wires:
  Product1/1 -> Add1/1
  Saturation/1 -> Product1/2, Product1/1
  w_thr/1 -> Add1/2
  In1/1 -> Saturation/1
  Sqrt/1 -> Out1/1
  Add1/1 -> Sqrt/1

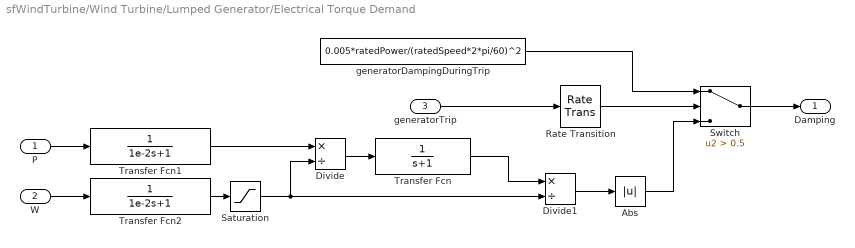
== system sfWindTurbine/Wind Turbine/Lumped Generator/Electrical Torque Demand ==
  P : Inport
  W : Inport  Port=2
  generatorTrip : Inport  Port=3
  Abs : Abs  SaturateOnIntegerOverflow=off
  Divide : Product  Inputs=*/
  Divide1 : Product  Inputs=*/
  Rate Transition : RateTransition
  Saturation : Saturate  UpperLimit=inf  LowerLimit=0.2*ratedSpeed*2*pi/60
  Switch : Switch  Criteria=u2 > Threshold  Threshold=0.5  SaturateOnIntegerOverflow=off  InputSameDT=off
  Transfer Fcn : TransferFcn  Denominator=[1 1]
  Transfer Fcn1 : TransferFcn  Denominator=[1e-2 1]
  Transfer Fcn2 : TransferFcn  Denominator=[1e-2 1]
  generatorDampingDuringTrip : Constant  Value=0.005*ratedPower/(ratedSpeed*2*pi/60)^2
  Damping : Outport
  wires:
  Rate Transition/1 -> Switch/2
  Divide1/1 -> Abs/1
  Divide/1 -> Transfer Fcn/1
  Transfer Fcn/1 -> Divide1/1
  W/1 -> Transfer Fcn2/1
  Transfer Fcn1/1 -> Divide/1
  P/1 -> Transfer Fcn1/1
  Transfer Fcn2/1 -> Saturation/1
  Saturation/1 -> Divide1/2, Divide/2
  generatorTrip/1 -> Rate Transition/1
  Abs/1 -> Switch/3
  Switch/1 -> Damping/1
  generatorDampingDuringTrip/1 -> Switch/1

== stateflow chart sfWindTurbine/Turbine State Machine ==
  settings: updateMethod=DISCRETE  sampleTime=0.01
  state Startup
    entry: StateMachineCMD.parkingBrake = OFF;
    StateMachineCMD.generatorTrip = ON;
    StateMachineCMD.pitchBrake = OFF;
    StateMachineCMD.turbineState = 1;
  state Generating
    entry: StateMachineCMD.parkingBrake = OFF;
    StateMachineCMD.generatorTrip = OFF;
    StateMachineCMD.pitchBrake = OFF;
    StateMachineCMD.turbineState = 2;
    StateMachineCMD.pitchROC =  20;
    exit: StateMachineCMD.powerGenState = 0;
    state MPPT
      entry: StateMachineCMD.powerGenState = 1;
    state ConstSpeed
      entry: StateMachineCMD.powerGenState = 2;
    state ConstPower
      entry: StateMachineCMD.powerGenState = 3;
    MPPT -> ConstSpeed : [duration(WindTurbineInput.WindSpeed>vWind_MaxGenSpeed_U)>0.1]
    ConstSpeed -> ConstPower [order 1] : [duration(WindTurbineInput.WindSpeed>vWind_RatedPower_U)>0.1]
    (default) -> MPPT
    ConstSpeed -> MPPT [order 2] : [duration(WindTurbineInput.WindSpeed<vWind_MaxGenSpeed_L)>0.1]
    ConstPower -> ConstSpeed : [duration(WindTurbineInput.WindSpeed<vWind_RatedPower_L)>0.1]
  state ParkBrake
    entry: StateMachineCMD.parkingBrake = ON;
    StateMachineCMD.generatorTrip = ON;
    StateMachineCMD.pitchBrake = OFF;
    StateMachineCMD.turbineState = 0;
  state PitchBrakeNormal
    entry: StateMachineCMD.parkingBrake = OFF;
    StateMachineCMD.generatorTrip = OFF;
    StateMachineCMD.pitchBrake = ON;
    StateMachineCMD.turbineState = 3;
    StateMachineCMD.pitchROC =  pitchROC_low;
  state PitchBrakeFast
    entry: StateMachineCMD.parkingBrake = OFF;
    StateMachineCMD.generatorTrip = ON;
    StateMachineCMD.pitchBrake = ON;
    StateMachineCMD.turbineState = 4;
    StateMachineCMD.pitchROC =  pitchROC_high;
  note: Higher tolerance to activate park break in case of emergency
  (junction 37) -> Startup : [duration(WindTurbineInput.WindSpeed>vWind_CutIn_L)>0.10...
      | &&duration(WindTurbineInput.WindSpeed<vWind_CutOut)>0.10...
      | && (EmergencyStop==0)...
      | &&NonEmergencyStop==0]
  Startup -> (junction 41) [order 1] : [duration(WindTurbineInput.wTurbine>...
      | turbine_speed_cut_in_U)>0.10]
  ParkBrake -> (junction 37)
  (junction 41) -> Generating
  Startup -> PitchBrakeNormal [order 2] : [duration(WindTurbineInput.WindSpeed<...
      | (vWind_CutIn_L))>1.0...
      | ||duration(WindTurbineInput.WindSpeed>...
      | vWind_CutOut)>1.0]
  PitchBrakeNormal -> Startup [order 2] : [duration(WindTurbineInput.WindSpeed<=...
      | vWind_CutIn_U)>2.0...
      | && duration(WindTurbineInput.WindSpeed>...
      | (vWind_CutIn_L))>2.0...
      | && duration(WindTurbineInput.wTurbine<...
      | turbine_speed_cut_in_U)>2.0]
  (default) -> ParkBrake
  (junction 39) -> ParkBrake
  Generating -> (junction 43) [order 1] : [duration(WindTurbineInput.WindSpeed<vWind_CutIn_L)>0.10...
      | ||duration(WindTurbineInput.WindSpeed>vWind_CutOut)>0.10...
      | ||duration(WindTurbineInput.wTurbine>turbine_speed_cut_out)>0.10...
      | ||duration(WindTurbineInput.wTurbine<turbine_speed_cut_in_L)>0.10...
      | ||NonEmergencyStop>0]
  Generating -> (junction 103) [order 2] : [EmergencyStop>0]
  (junction 43) -> PitchBrakeNormal
  PitchBrakeNormal -> (junction 39) [order 1] : [duration(WindTurbineInput.wTurbine<=...
      | park_speed)>0.10]
  (junction 108) -> (junction 39)
  PitchBrakeNormal -> PitchBrakeFast [order 3] : [EmergencyStop>0]
  PitchBrakeFast -> (junction 108) : [duration(WindTurbineInput.wTurbine<=...
      | (park_speed*18))>0.10]
  (junction 103) -> PitchBrakeFast
  data: turbine_speed_cut_in_L local double =wTurbineCutIn_L; vWind_CutOut local double =vWindCutOut; vWind_CutIn_U local double =vWindCutIn_U; turbine_speed_cut_out local double =wTurbineCutOut; park_speed constant double =wTurbinePark; vWind_RatedPower_L local double =vWindRatedPower_L; vWind_MaxGenSpeed_L local double =vWindMaxGenSpeed_L; vWind_RatedPower_U local double =vWindRatedPower_U; vWind_MaxGenSpeed_U local double =vWindMaxGenSpeed_U; vWind_CutIn_L local double =vWindCutIn_L; turbine_speed_cut_in_U local double =wTurbineCutIn_U; EmergencyStop input; NonEmergencyStop input; StateMachineCMD output Bus: StateMachineBus; WindTurbineInput input Bus: WindTurbineBus; pitchROC_low constant double =5; pitchROC_high constant double =20; ON constant double =1; OFF local double =0
